simulink model "NIBB_Single"  (R2022a)
settings: Solver=VariableStepAuto  StartTime=0.0  StopTime=1  RelTol=1e-3
libraries: spsSeriesRLCBranchLib x3, spsCurrentMeasurementLib x2, spsDiodeLib x2, spsMosfetLib x2, spsVoltageMeasurementLib x2, spsDCVoltageSourceLib x1, spspowerguiLib x1
settings Model: Creator=Bobby  LastModifiedBy=Bobby

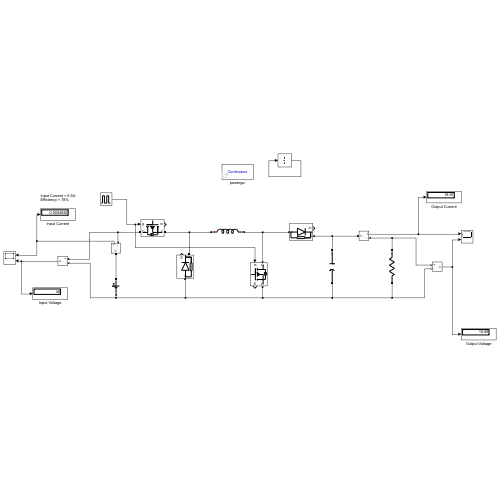
[thumbnail: Simulink's stored preview of the top-level diagram]
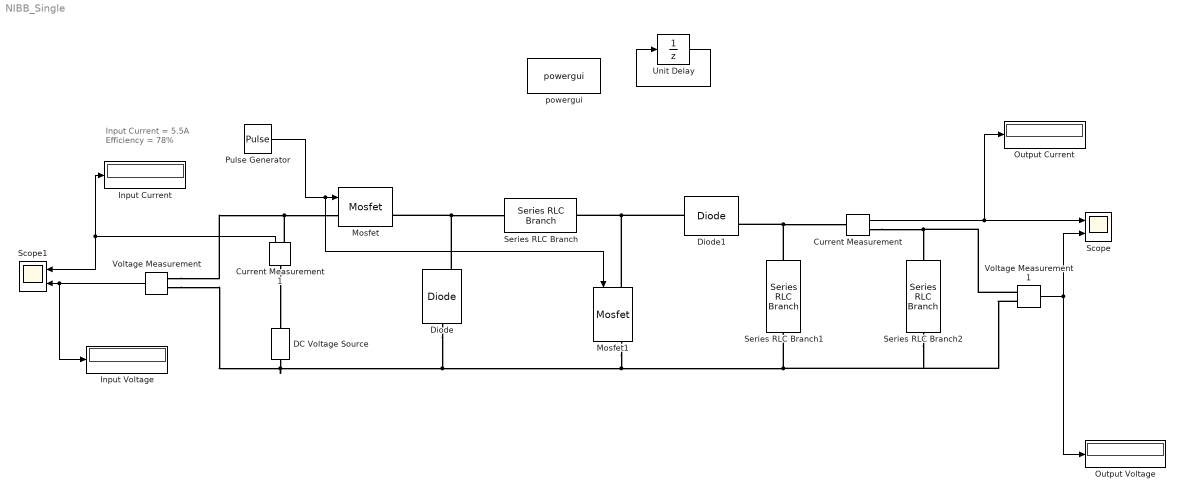
== system NIBB_Single ==
  note: Input Current = 5.5A
      | Efficiency = 78%
  Current Measurement : spsCurrentMeasurementLib/Current Measurement  PhasorSimulation=off  OutputType=Complex  PSBequivalent=0
  Current Measurement1 : spsCurrentMeasurementLib/Current Measurement  PhasorSimulation=off  OutputType=Complex  PSBequivalent=0
  DC Voltage Source : spsDCVoltageSourceLib/DC Voltage Source  Amplitude=48  Measurements=None
  Diode : spsDiodeLib/Diode  Ron=0.001  Lon=0  Vf=0.8  IC=0  UseSnubber=0  Rs=500  Cs=250e-9  Measurements=on
  Diode1 : spsDiodeLib/Diode  Ron=0.001  Lon=0  Vf=0.8  IC=0  UseSnubber=0  Rs=500  Cs=250e-9  Measurements=on
  Input Current : Display
  Input Voltage : Display
  Mosfet : spsMosfetLib/Mosfet  Ron=0.1  Lon=0  Rd=0.01  Vfd=0  IC=0  Rs=1e5  Cs=inf  Measurements=on
  Mosfet1 : spsMosfetLib/Mosfet  Ron=0.1  Lon=0  Rd=0.01  Vfd=0  IC=0  Rs=1e5  Cs=inf  Measurements=on
  Output Current : Display
  Output Voltage : Display
  Pulse Generator : DiscretePulseGenerator  PulseType=Time based  Period=20e-6  PulseWidth=22.5
  Scope : Scope  NumInputPorts=2
  Scope1 : Scope  NumInputPorts=2
  Series RLC Branch : spsSeriesRLCBranchLib/Series RLC Branch  LConnTagsString=__new0  RConnTagsString=__new0  BranchType=L  Resistance=1  Inductance=30e-6  SetiL0=off  InitialCurrent=0  Capacitance=1e-6  Setx0=off  InitialVoltage=0  Measurements=None
  Series RLC Branch1 : spsSeriesRLCBranchLib/Series RLC Branch  LConnTagsString=__new0  RConnTagsString=__new0  BranchType=C  Resistance=1  Inductance=1e-3  SetiL0=off  InitialCurrent=0  Capacitance=1664e-6  Setx0=off  InitialVoltage=0  Measurements=None
  Series RLC Branch2 : spsSeriesRLCBranchLib/Series RLC Branch  LConnTagsString=__new0  RConnTagsString=__new0  BranchType=R  Resistance=0.576  Inductance=1e-3  SetiL0=off  InitialCurrent=0  Capacitance=1e-6  Setx0=off  InitialVoltage=0  Measurements=None
  Unit Delay : UnitDelay  SampleTime=-1  HasFrameUpgradeWarning=on
  Voltage Measurement : spsVoltageMeasurementLib/Voltage Measurement  PhasorSimulation=off  OutputType=Complex  PSBequivalent=0
  Voltage Measurement1 : spsVoltageMeasurementLib/Voltage Measurement  PhasorSimulation=off  OutputType=Complex  PSBequivalent=0
  powergui : spspowerguiLib/powergui  Priority=1  SimulationMode=Continuous  SampleTime=50e-6  frequency=60  Iterations=50  frequencyindice=0  Pbase=100e6  ErrMax=1e-4  UnitsV=kV  UnitsW=MW  buscounter=0  FunctionMessages=off  echomessages=off  EnableUseOfTLC=off  CurrentSourceSwitches=off  DisableSnubberDevices=off  DisableRonSwitches=off  DisableVfSwitches=off  DisplayEquations=off  AutomaticDiscreteSolvers=off  SolverType=Tustin/Backward Euler (TBE)  Interpol=off  ExternalGateDelay=off  methode=off  Ts=100  x0status=blocks  SPID=on  SwTol=0  HookPort=off  NonlinearTolerance=1e-4  nMaxIteration=100  ContinueOnMaxIteration=off  RestoreLinks=warning  ResistiveCurrentMeasurement=off  Frange=[0:2:500]  Ylog=off  Xlog=on  ShowGrid=off  save=off  variable=ZData  structure=0  ZoomFFT=off  StartTime=0.0  cycles=1  DisplayStyle=1  fundamental=60  FreqAxis=off  MaxFrequency=1000  frequencyindicesteady=1  RmsSteady=1  display=off
  wires:
  Pulse Generator/1 -> Mosfet1/1, Mosfet/1
  Voltage Measurement1/1 -> Output Voltage/1, Scope/2
  Current Measurement/1 -> Output Current/1, Scope/1
  Voltage Measurement/1 -> Input Voltage/1, Scope1/2
  Current Measurement1/1 -> Input Current/1, Scope1/1
  Unit Delay/1 -> Unit Delay/1
  connections:
  Diode/RConn1 -- Series RLC Branch/LConn1 -- Mosfet/RConn1
  Mosfet1/LConn1 -- Series RLC Branch/RConn1 -- Diode1/LConn1
  Series RLC Branch1/LConn1 -- Current Measurement/LConn1 -- Diode1/RConn1
  DC Voltage Source/LConn1 -- Voltage Measurement/LConn2 -- Diode/LConn1 -- Mosfet1/RConn1 -- Series RLC Branch2/RConn1 -- Voltage Measurement1/LConn2 -- Series RLC Branch1/RConn1
  Current Measurement/RConn1 -- Voltage Measurement1/LConn1 -- Series RLC Branch2/LConn1
  Voltage Measurement/LConn1 -- Current Measurement1/RConn1 -- Mosfet/LConn1
  Current Measurement1/LConn1 -- DC Voltage Source/RConn1
